simulink model "vsi_01_open_loop"  (R2026a)
settings: Solver=FixedStepDiscrete  StopTime=Tstop  FixedStep=Ts
PostLoadFcn:
  | run(fullfile(fileparts(get_param('vsi_01_open_loop','FileName')), 'params_01_open_loop.m'));
InitFcn:
  | run(fullfile(fileparts(get_param('vsi_01_open_loop','FileName')), 'params_01_open_loop.m'));
values from neighbouring files (symbols this model uses):
  delta = angle(E_ph)    [params_01_open_loop.m]
  Lf = 5e-3    (= 0.005)    [params_01_open_loop.m]
  Lg = 1e-3    (= 0.001)    [params_01_open_loop.m]
  Rf = 0.5    [params_01_open_loop.m]
  Rg = 0.1    [params_01_open_loop.m]
  tau_pq = 5e-3    (= 0.005)    [params_01_open_loop.m]
  Ts = 1e-6    (= 1e-06)    [params_01_open_loop.m]
  Vdc = 700    [params_01_open_loop.m]
  Vinv_pk = sqrt(2)*abs(E_ph)    [params_01_open_loop.m]
  wg = 2*pi*fg    (= 314.159265359)    [params_01_open_loop.m]
libraries: nesl_utility x9, ee_lib x5, fl_lib x2, eePwmGeneratorTwoLevel x1
settings Model: Creator=HAKAN SARI  LastModifiedBy=HAKAN SARI
settings SimscapeCC: SimscapeLogType=none

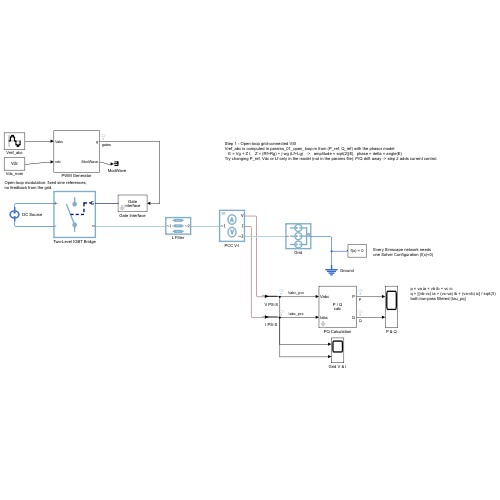
[thumbnail: Simulink's stored preview of the top-level diagram]
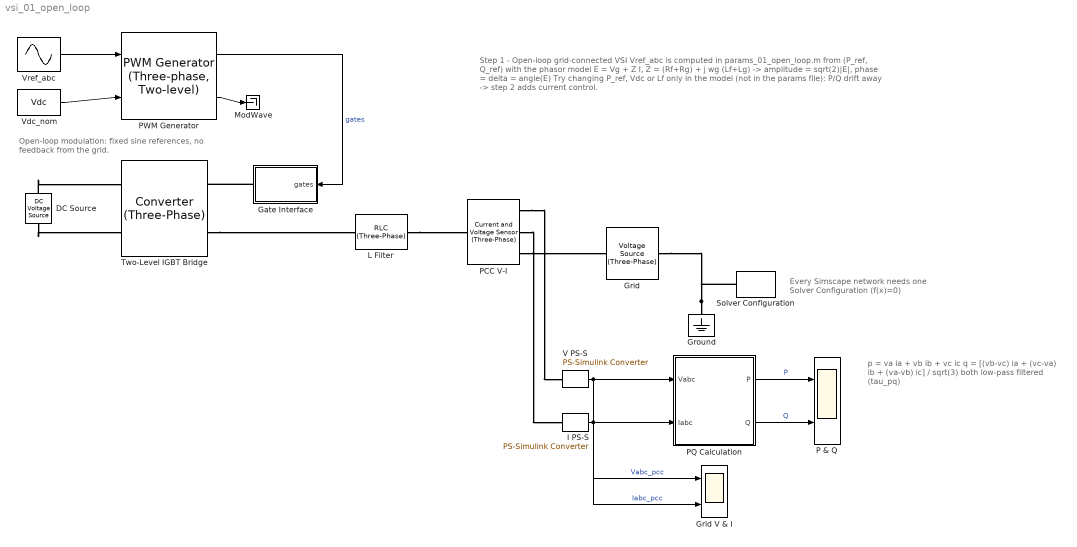
== system vsi_01_open_loop ==
  note: Step 1 - Open-loop grid-connected VSI
      | Vref_abc is computed in params_01_open_loop.m from (P_ref, Q_ref) with the phasor model
      |    E = Vg + Z I,   Z = (Rf+Rg) + j wg (Lf+Lg)   ->   amplitude = sqrt(2)|E|,  phase = delta = angle(E)
      | Try changing P_ref, Vdc or Lf only in the model (not in the params file): P/Q drift away -> step 2 adds current control.
  note: Every Simscape network needs
      | one Solver Configuration (f(x)=0)
  note: Open-loop modulation: fixed sine references,
      | no feedback from the grid.
  note: p = va ia + vb ib + vc ic
      | q = [(vb-vc) ia + (vc-va) ib + (va-vb) ic] / sqrt(3)
      | both low-pass filtered (tau_pq)
  DC Source : fl_lib/Electrical/Electrical Sources/DC Voltage Source  v0=Vdc V
  Gate Interface : Subsystem
      mask help: Converts the boolean PWM gate vector [a+ a- b+ b- c+ c-] into the converter gate port (Q1..Q6).
      mask Display: disp('Gate\ninterface');
  Grid : ee_lib/Sources/Voltage Source (Three-Phase)  vline_rms=Vg_ll V  shift=0 deg  freq=fg Hz  impedance_option=4  SShortCircuit=1e6 A*V  XR=15  R=Rg Ohm  L=Lg H  harmonic_option=0  harmonic_orders=[5, 7, 11, 13]  harmonic_ratios=[.1, .1, .1, .1]  G_parasitic=0 1/Ohm  I_specify=off  I_priority=None  I=[0, 0, 0] A  I_nominal_specify=off  I_nominal_value=1  I_nominal_unit=A
  Grid V & I : Scope  NumInputPorts=2
  Ground : fl_lib/Electrical/Electrical Elements/Electrical Reference
  I PS-S : nesl_utility/PS-Simulink Converter  PhysicalDomain=network_engine_domain  SubClassName=ps_output  LeftPortType=input  RightPortType=output  PseudoPeriodic=off  Frequencies=[]  VectorFormat=1-D array  Unit=inherit  AffineConversion=off
  L Filter : ee_lib/Passive/RLC Assemblies/RLC (Three-Phase)  port_option=ee.enum.threePhasePort.composite  component_structure=4  R=Rf Ohm  L=Lf H  C=1e-6 F  R_parasitic=0 Ohm  G_parasitic=0 1/Ohm  IL_specify=off  IL_priority=High  IL=[0, 0, 0] A  IL_nominal_specify=off  IL_nominal_value=1  IL_nominal_unit=A  VC_specify=off  VC_priority=High  VC=[0, 0, 0] V  VC_nominal_specify=off  VC_nominal_value=1  VC_nominal_unit=V
  ModWave : Terminator
  P & Q : Scope  NumInputPorts=2
  PCC V-I : ee_lib/Sensors & Transducers/Current and Voltage Sensor (Three-Phase)  port_option=ee.enum.threePhasePort.composite  vMeasurementType=2  outputUnit=2  SRated=100e6 A*V  VRated=24e3 V  I_specify=off  I_priority=None  I=[0, 0, 0] A  I_nominal_specify=off  I_nominal_value=1  I_nominal_unit=A  V_specify=off  V_priority=None  V=[0, 0, 0] V  V_nominal_specify=off  V_nominal_value=1  V_nominal_unit=V
  PQ Calculation : Subsystem
      mask help: Instantaneous three-phase active/reactive power with first-order low-pass filter.
      mask Display: port_label('input',1,'Vabc');port_label('input',2,'Iabc');port_label('output',1,'P');port_label('output',2,'Q');disp('P / Q\ncalc');
  PWM Generator : eePwmGeneratorTwoLevel/PWM Generator (Three-phase, Two-level)  PWMMode=Continuous PWM (CPWM)  CPWMMode=SPWM: sinusoidal PWM  DPWMMode=60 DPWM: 60 degree discontinuous PWM  fsw=fsw  Ts=Ts
  Solver Configuration : nesl_utility/Solver Configuration  PhysicalDomain=network_engine_domain  SubClassName=solver  LeftPortType=input  RightPortType=generic  Tones=[]  Harmonics=[]  SimulateNoise=off  Profile=off  UseLocalSampling=off  EnableSwitchedLinearOptims=on  FrequencyDomain=off  UseCCode=off  RelTol=0.001  AbsTol=0.001  MinStep=1e-09  ToWorkspace=off  RevertToSquareIcSolve=off  NumHomotopyIterations=100  PhasorMode=off  PhasorModeNumHarmonics=1  ConsistencySolver=NEWTON_XTOL_AFTER_FTOL  CanonicalOrdering=CANONICAL  OptimizeIntermediates=OPTIMIZED  IndexReductionMethod=DerivativeReplacement  DoDC=off  ResidualTolerance=1e-09  ConsistencyTolSource=GLOBAL  ConsistencyAbsTol=0.001  ConsistencyRelTol=0.001  ConsistencyTolFactor=0.001  UseLocalSolver=on  LocalSolverChoice=NE_BACKWARD_EULER_ADVANCER  ResolveIndetEquations=on  FunctionEvalNumThread=1  LocalSolverSampleTime=Ts  DoFixedCost=off  MaxNonlinIter=3  MaxModeIter=2  ComputeImpulses=off  ImpulseIterations=2  LinearAlgebra=auto  LinearAlgebraNumThread=0  EquationFormulation=NE_TIME_EF  DelaysMemoryBudget=1024  AutomaticFiltering=on  FilteringTimeConstant=0.001  PartitionStorageMethod=AS_NEEDED  PartitionMemoryBudget=1024  PartitionMethod=ROBUST  MultibodyUseLocalSolver=off  MultibodyLocalSolverChoice=ODE1  MultibodyLocalSolverSampleTime=0.001
  Two-Level IGBT Bridge : ee_lib/Semiconductors & Converters/Converters/Converter (Three-Phase)  port_option=ee.enum.threePhasePort.composite  fidelity_option=ee.enum.converters.fidelity.detailed  device_type=ee.enum.converters.switchingdevice.igbt  showThermalPort=false  K=0  Vth=0.5 V  Vgt=1 V  Vgt_off=-1 V  Ih=1 A  Vf=Vf_sw V  Ron=Ron_sw Ohm  Rds=0.001 Ohm  Goff=1e-6 1/Ohm  Eon_scalar=22.86e-3 J  Eoff_scalar=17.14e-3 J  Eoff_natural_commutation=10e-3 J  Voff=300 V  Iout_scalar=600 A  onCurrentMeasDelay=0 s  useCurrentFromPreviousCycle=false  useVoltageFromPreviousCycle=false  diode_param=ee.enum.converters.protectiondiode.nodynamics  diode_Vf=Vf_sw V  diode_Ron=Ron_sw Ohm  diode_Goff=1e-6 1/Ohm  diode_C=50 nF  diode_iRM=-235 A  diode_iF=300 A  diode_idot=-50 A/us  diode_trr_param=ee.enum.converters.diodetrr.trr_factor  diode_trr_factor=3  diode_trr=15 us  diode_Qrr=1500 s*uA  diode_rec_loss_model=ee.enum.diode.reverseRecoveryModel.fixed  diode_ErecVal=0 J  diode_scaleWithIandV=false  diode_ErecMat=zeros(2, 3) J  diode_TjrecVec=[298.15, 398.15] K  diode_IfrecVec=[.1, 1, 10] A  diode_IrecVal=10 A  diode_VrecVal=10 V  diode_tFilter=1 / 1000 / 100 s  thermal_network_parameterization=ee.enum.thermalNetworkTopology.external  Rth=[.08, .5] K/W  Rth_Cauer=[.08, .1, .5] K/W  Rth_Foster=[.08, .14, .22, .16] K/W  thermal_mass_parameterization=ee.enum.thermalNetwork.timeconstant  thermal_mass=[.01, .5] J/K  thermal_mass_Cauer=[.01, .1, .5] J/K  thermal_mass_Foster=[.001, .005, .05, .5] J/K  thermal_time_constant=[.001, .2] s  thermal_time_constant_Cauer=[.001, .1, .2] s  thermal_time_constant_Foster=[7e-05, .0007, .01, .08] s  thermal_mass_initial_temperatures=[25, 25] degC  thermal_mass_initial_temperatures_Cauer=[25, 25, 25] degC  junction_thermal_mass=0.01 J/K  Tvec_initial_Foster=[25, 25, 25, 25] degC  snubber_type=0  Cs=1e-7 F  Rs=0.1 Ohm  Vce_loss=[0, 150, 300] V
  V PS-S : nesl_utility/PS-Simulink Converter  PhysicalDomain=network_engine_domain  SubClassName=ps_output  LeftPortType=input  RightPortType=output  PseudoPeriodic=off  Frequencies=[]  VectorFormat=1-D array  Unit=inherit  AffineConversion=off
  Vdc_nom : Constant  Value=Vdc  SampleTime=Ts
  Vref_abc : Sin  Amplitude=Vinv_pk  Frequency=wg  Phase=[delta, delta-2*pi/3, delta+2*pi/3]  SampleTime=Ts
  wires:
  Vref_abc/1 -> PWM Generator/1
  Vdc_nom/1 -> PWM Generator/2
  PWM Generator/2 -> ModWave/1
  PWM Generator/1 -> Gate Interface/1(gates)  "gates"
  V PS-S/1 -> PQ Calculation/1(Vabc), Grid V & I/1  "Vabc_pcc"
  I PS-S/1 -> PQ Calculation/2(Iabc), Grid V & I/2  "Iabc_pcc"
  PQ Calculation/1(P) -> P & Q/1  "P"
  PQ Calculation/2(Q) -> P & Q/2  "Q"
  connections:
  DC Source/LConn1 -- Two-Level IGBT Bridge/RConn1
  DC Source/RConn1 -- Two-Level IGBT Bridge/RConn2
  Two-Level IGBT Bridge/LConn2 -- L Filter/LConn1
  L Filter/RConn1 -- PCC V-I/LConn1
  PCC V-I/RConn3 -- Grid/RConn1
  Ground/LConn1 -- Grid/LConn1 -- Solver Configuration/RConn1
  Gate Interface/RConn1 -- Two-Level IGBT Bridge/LConn1
  PCC V-I/RConn1 -- V PS-S/LConn1
  PCC V-I/RConn2 -- I PS-S/LConn1

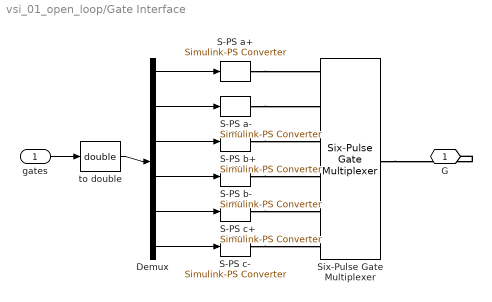
== system vsi_01_open_loop/Gate Interface ==
  gates : Inport
  Demux : Demux  Outputs=6
  S-PS a+ : nesl_utility/Simulink-PS Converter  PhysicalDomain=network_engine_domain  SubClassName=ps_input  LeftPortType=input  RightPortType=output  PseudoPeriodic=off  Frequencies=[]  NoiseDistribution=none  NoiseParameters=[]  Unit=1  AffineConversion=off  FilteringAndDerivatives=zero  SimscapeFilterOrder=1  InputFilterTimeConstant=0.001  UdotUserProvided=0
  S-PS a- : nesl_utility/Simulink-PS Converter  PhysicalDomain=network_engine_domain  SubClassName=ps_input  LeftPortType=input  RightPortType=output  PseudoPeriodic=off  Frequencies=[]  NoiseDistribution=none  NoiseParameters=[]  Unit=1  AffineConversion=off  FilteringAndDerivatives=zero  SimscapeFilterOrder=1  InputFilterTimeConstant=0.001  UdotUserProvided=0
  S-PS b+ : nesl_utility/Simulink-PS Converter  PhysicalDomain=network_engine_domain  SubClassName=ps_input  LeftPortType=input  RightPortType=output  PseudoPeriodic=off  Frequencies=[]  NoiseDistribution=none  NoiseParameters=[]  Unit=1  AffineConversion=off  FilteringAndDerivatives=zero  SimscapeFilterOrder=1  InputFilterTimeConstant=0.001  UdotUserProvided=0
  S-PS b- : nesl_utility/Simulink-PS Converter  PhysicalDomain=network_engine_domain  SubClassName=ps_input  LeftPortType=input  RightPortType=output  PseudoPeriodic=off  Frequencies=[]  NoiseDistribution=none  NoiseParameters=[]  Unit=1  AffineConversion=off  FilteringAndDerivatives=zero  SimscapeFilterOrder=1  InputFilterTimeConstant=0.001  UdotUserProvided=0
  S-PS c+ : nesl_utility/Simulink-PS Converter  PhysicalDomain=network_engine_domain  SubClassName=ps_input  LeftPortType=input  RightPortType=output  PseudoPeriodic=off  Frequencies=[]  NoiseDistribution=none  NoiseParameters=[]  Unit=1  AffineConversion=off  FilteringAndDerivatives=zero  SimscapeFilterOrder=1  InputFilterTimeConstant=0.001  UdotUserProvided=0
  S-PS c- : nesl_utility/Simulink-PS Converter  PhysicalDomain=network_engine_domain  SubClassName=ps_input  LeftPortType=input  RightPortType=output  PseudoPeriodic=off  Frequencies=[]  NoiseDistribution=none  NoiseParameters=[]  Unit=1  AffineConversion=off  FilteringAndDerivatives=zero  SimscapeFilterOrder=1  InputFilterTimeConstant=0.001  UdotUserProvided=0
  Six-Pulse Gate Multiplexer : ee_lib/Semiconductors & Converters/Converters/Six-Pulse Gate Multiplexer  port_option=ee.enum.controlport.ps
  to double : DataTypeConversion  OutDataTypeStr=double  SaturateOnIntegerOverflow=off  RndMeth=Floor
  G : PMIOPort  Side=Right
  wires:
  gates/1 -> to double/1
  to double/1 -> Demux/1
  Demux/1 -> S-PS a+/1
  Demux/2 -> S-PS a-/1
  Demux/3 -> S-PS b+/1
  Demux/4 -> S-PS b-/1
  Demux/5 -> S-PS c+/1
  Demux/6 -> S-PS c-/1
  connections:
  S-PS a+/RConn1 -- Six-Pulse Gate Multiplexer/LConn1
  S-PS a-/RConn1 -- Six-Pulse Gate Multiplexer/LConn2
  S-PS b+/RConn1 -- Six-Pulse Gate Multiplexer/LConn3
  S-PS b-/RConn1 -- Six-Pulse Gate Multiplexer/LConn4
  S-PS c+/RConn1 -- Six-Pulse Gate Multiplexer/LConn5
  S-PS c-/RConn1 -- Six-Pulse Gate Multiplexer/LConn6
  Six-Pulse Gate Multiplexer/RConn1 -- G/RConn1

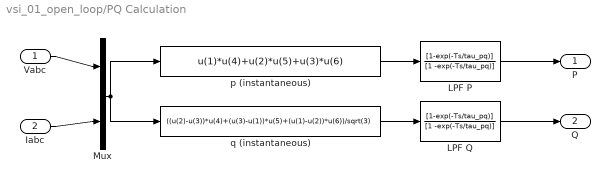
== system vsi_01_open_loop/PQ Calculation ==
  Vabc : Inport
  Iabc : Inport  Port=2
  LPF P : DiscreteTransferFcn  Numerator=[1-exp(-Ts/tau_pq)]  Denominator=[1 -exp(-Ts/tau_pq)]  SampleTime=Ts
  LPF Q : DiscreteTransferFcn  Numerator=[1-exp(-Ts/tau_pq)]  Denominator=[1 -exp(-Ts/tau_pq)]  SampleTime=Ts
  Mux : Mux  Inputs=2
  p (instantaneous) : Fcn  Expr=u(1)*u(4)+u(2)*u(5)+u(3)*u(6)
  q (instantaneous) : Fcn  Expr=((u(2)-u(3))*u(4)+(u(3)-u(1))*u(5)+(u(1)-u(2))*u(6))/sqrt(3)
  P : Outport
  Q : Outport  Port=2
  wires:
  Vabc/1 -> Mux/1
  Iabc/1 -> Mux/2
  Mux/1 -> p (instantaneous)/1, q (instantaneous)/1
  p (instantaneous)/1 -> LPF P/1
  q (instantaneous)/1 -> LPF Q/1
  LPF P/1 -> P/1
  LPF Q/1 -> Q/1
